simulink model "EvitarObstaculo_traj"  (R2023b)
settings: Solver=FixedStepAuto  StartTime=0.0  StopTime=100.0  FixedStep=Ts  RelTol=1e-3
values from neighbouring files (symbols this model uses):
  obsx = 2    [EjecutarEsquivarObs.m]    (also in EjecutarEsquivarObs_traj.m = 1.75)
  obsy = 0    [EjecutarEsquivarObs.m]    (also in EjecutarEsquivarObs_traj.m = 0.7)
  th_0 = 0    [EjecutarBorroso_traj.m]    (also in EjecutarEsquivarObs_traj.m)
  Ts = 100e-3    (= 0.1)    [EjecutarBorroso.m]    (also in EjecutarBorroso_traj.m; EjecutarEsquivarObs.m; EjecutarEsquivarObs_traj.m)
  x_0 = 0.1    [EjecutarBorroso_traj.m]    (also in EjecutarEsquivarObs_traj.m)
  y_0 = 0    [EjecutarBorroso_traj.m]    (also in EjecutarEsquivarObs_traj.m)
undefined symbols (not defined in the file or in its folder): DiscIntNeverNeededParam, sigbuilder_block
libraries: fuzblock x1
settings Model: Creator=perez  LastModifiedBy=perez
settings DataIOCC: ReturnWorkspaceOutputs=off

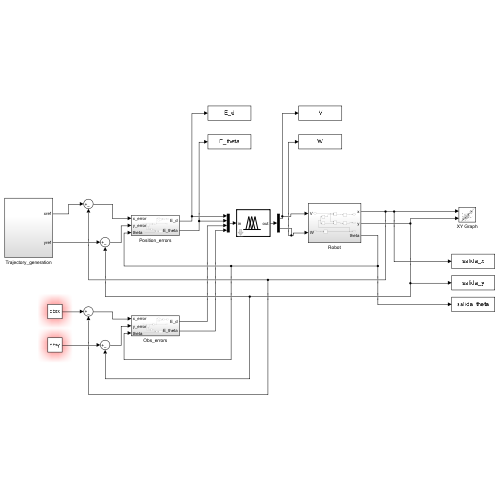
[thumbnail: Simulink's stored preview of the top-level diagram]
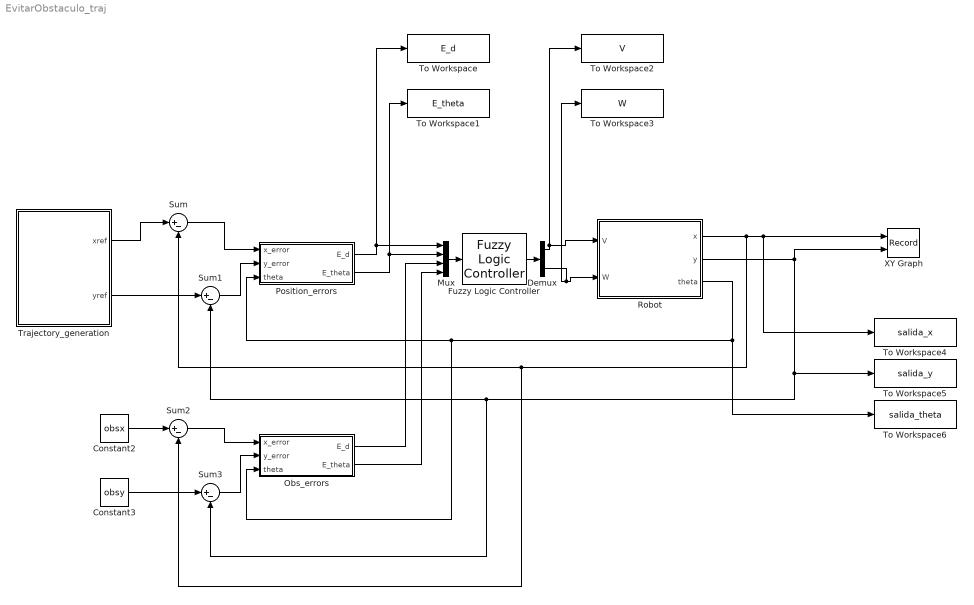
== system EvitarObstaculo_traj ==
  Constant2 : Constant  Value=obsx
  Constant3 : Constant  Value=obsy
  Demux : Demux  Outputs=2
  Fuzzy Logic Controller : fuzblock/Fuzzy Logic  Controller  FIS='ControlBorrosoObs.fis'  OutputSampleNumber=101  DataType=double  FuzzifiedInputs=off  RuleFiringStrengths=off  RuleOutputs=off  AggregatedOutputs=off  SimulateUsing=Interpreted execution  OutOfRangeInputValueMessage=warning  NoRuleFiredMessage=warning  EmptyOutputFuzzySetMessage=warning
  Mux : Mux
  Obs_errors : Subsystem
  Position_errors : Subsystem
  Robot : Subsystem
  Sum{,1..3} (4 alike) : Sum  Inputs=|+-
  To Workspace : ToWorkspace  VariableName=E_d  SaveFormat=Structure With Time  SampleTime=-1
  To Workspace1 : ToWorkspace  VariableName=E_theta  SaveFormat=Structure With Time  SampleTime=-1
  To Workspace2 : ToWorkspace  VariableName=V  SaveFormat=Structure With Time  SampleTime=-1
  To Workspace3 : ToWorkspace  VariableName=W  SaveFormat=Structure With Time  SampleTime=-1
  To Workspace4 : ToWorkspace  VariableName=salida_x  SaveFormat=Structure With Time  SampleTime=-1
  To Workspace5 : ToWorkspace  VariableName=salida_y  SaveFormat=Structure With Time  SampleTime=-1
  To Workspace6 : ToWorkspace  VariableName=salida_theta  SaveFormat=Structure With Time  SampleTime=-1
  Trajectory_generation : Subsystem
  XY Graph : Record  FileSettingsInternal="{\"entries\":[{\"content\":{\"excelSettings\":{\"content\":{},\"type\":\"Streamout.ExcelSettings\"}},\"type\":\"Streamout.FileSettingStorage\",\"uuid\":\"\"}],\"packageUris\":[\"http:\\/\\/schema.mathworks.com\\/mf0\\/streamout_blocks\\/R2020a\"],\"version\":\"1.0\"}"  Layout=[1 1]  SignalsInternal="{\"entries\":[{\"content\":{\"signals\":[{\"content\":{\"blockPath\":[],\"dimensions\":[1],\"domain\":\"\",\"lineColor\":\"#a2142f\",\"plots\":[ 1 ],\"port\":1,\"signalID\":1,\"signalName\":\"Robot:1\"},\"type\":\"RecordBlkView.Signal\",\"uuid\":\"\"},{\"content\":{\"blockPath\":[],\"dimensions\":[1],\"domain\":\"\",\"lineColor\":\"#139fff\",\"plots\":[ 1 ],\"port\":2,\"signalID\":2,\"signalName\":\"Robot:2\"},\"type\":\"RecordBlkView.Signal\",\"uuid\":\"\"}]},\"type\":\"RecordBlkView.InputSignals\",\"uuid\":\"\"}],\"packageUris\":[\"http:\\/\\/schema.mathworks.com\\/mf0\\/streamout_blocks\\/R2020a\"],\"version\":\"1.0\"}"  VisualizationBindings="{\"xyplotplugin\":{\"info\":[{\"series\":[{\"bindingParametersList\":[{\"parameter\":\"X-Axis\",\"signalID\":1,\"signalName\":\"Robot:1\"},{\"parameter\":\"Y-Axis\",\"signalID\":2,\"signalName\":\"Robot:2\"}],\"seriesID\":0}],\"subplotID\":1}]}}"  CompatibilityTag=XY
  wires:
  Trajectory_generation/1(xref) -> Sum/1
  Sum/1 -> Position_errors/1(x_error)
  Sum1/1 -> Position_errors/2(y_error)
  Position_errors/1(E_d) -> Mux/1, To Workspace/1
  Position_errors/2(E_theta) -> Mux/2, To Workspace1/1
  Demux/1 -> To Workspace2/1, Robot/1(V)
  Demux/2 -> To Workspace3/1, Robot/2(W)
  Robot/1(x) -> Sum2/2, Sum/2, To Workspace4/1, XY Graph/1
  Robot/2(y) -> To Workspace5/1, Sum3/2, Sum1/2, XY Graph/2
  Robot/3(theta) -> To Workspace6/1, Obs_errors/3(theta), Position_errors/3(theta)
  Trajectory_generation/2(yref) -> Sum1/1
  Mux/1 -> Fuzzy Logic Controller/1
  Fuzzy Logic Controller/1 -> Demux/1
  Constant2/1 -> Sum2/1
  Constant3/1 -> Sum3/1
  Sum2/1 -> Obs_errors/1(x_error)
  Sum3/1 -> Obs_errors/2(y_error)
  Obs_errors/1(E_d) -> Mux/3
  Obs_errors/2(E_theta) -> Mux/4

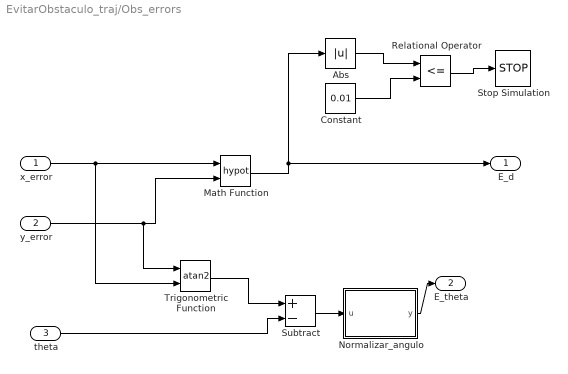
== system EvitarObstaculo_traj/Obs_errors ==
  x_error : Inport
  y_error : Inport  Port=2
  theta : Inport  Port=3
  Abs : Abs  SaturateOnIntegerOverflow=off
  Constant : Constant  Value=0.01
  Math Function : Math  Operator=hypot
  Normalizar_angulo : MATLAB Function  TreatAsAtomicUnit=on
  Relational Operator : RelationalOperator  Operator=<=  OutDataTypeStr=boolean  RndMeth=Simplest  InputSameDT=off
  Stop Simulation : Stop
  Subtract : Sum  Inputs=+-
  Trigonometric Function : Trigonometry  Operator=atan2
  E_d : Outport
  E_theta : Outport  Port=2
  wires:
  x_error/1 -> Trigonometric Function/2, Math Function/1
  y_error/1 -> Trigonometric Function/1, Math Function/2
  Trigonometric Function/1 -> Subtract/1
  theta/1 -> Subtract/2
  Subtract/1 -> Normalizar_angulo/1(u)
  Normalizar_angulo/1(y) -> E_theta/1
  Abs/1 -> Relational Operator/1
  Constant/1 -> Relational Operator/2
  Math Function/1 -> E_d/1, Abs/1
  Relational Operator/1 -> Stop Simulation/1

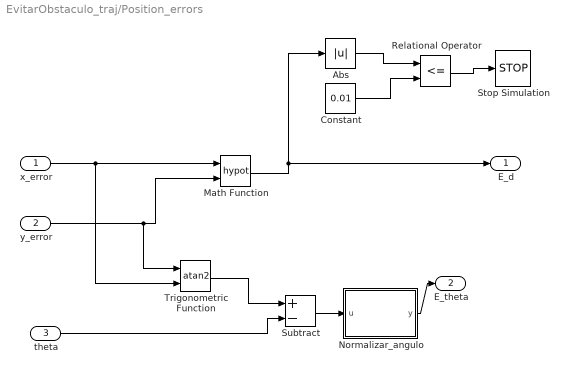
== system EvitarObstaculo_traj/Position_errors ==
  x_error : Inport
  y_error : Inport  Port=2
  theta : Inport  Port=3
  Abs : Abs  SaturateOnIntegerOverflow=off
  Constant : Constant  Value=0.01
  Math Function : Math  Operator=hypot
  Normalizar_angulo : MATLAB Function  TreatAsAtomicUnit=on
  Relational Operator : RelationalOperator  Operator=<=  OutDataTypeStr=boolean  RndMeth=Simplest  InputSameDT=off
  Stop Simulation : Stop
  Subtract : Sum  Inputs=+-
  Trigonometric Function : Trigonometry  Operator=atan2
  E_d : Outport
  E_theta : Outport  Port=2
  wires:
  x_error/1 -> Trigonometric Function/2, Math Function/1
  y_error/1 -> Trigonometric Function/1, Math Function/2
  Trigonometric Function/1 -> Subtract/1
  theta/1 -> Subtract/2
  Subtract/1 -> Normalizar_angulo/1(u)
  Normalizar_angulo/1(y) -> E_theta/1
  Abs/1 -> Relational Operator/1
  Constant/1 -> Relational Operator/2
  Math Function/1 -> E_d/1, Abs/1
  Relational Operator/1 -> Stop Simulation/1

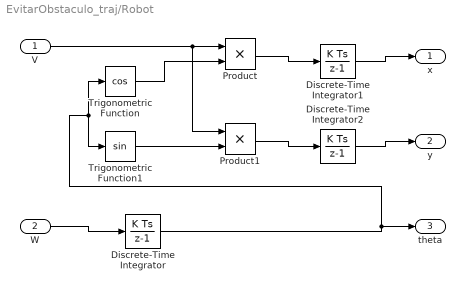
== system EvitarObstaculo_traj/Robot ==
  V : Inport
  W : Inport  Port=2
  Discrete-Time Integrator : DiscreteIntegrator  SampleTime=-1  ICPrevOutput=DiscIntNeverNeededParam  ICPrevScaledInput=DiscIntNeverNeededParam
  Discrete-Time Integrator1 : DiscreteIntegrator  SampleTime=-1  ICPrevOutput=DiscIntNeverNeededParam  ICPrevScaledInput=DiscIntNeverNeededParam
  Discrete-Time Integrator2 : DiscreteIntegrator  SampleTime=-1  ICPrevOutput=DiscIntNeverNeededParam  ICPrevScaledInput=DiscIntNeverNeededParam
  Product : Product
  Product1 : Product
  Trigonometric Function : Trigonometry  Operator=cos
  Trigonometric Function1 : Trigonometry
  x : Outport
  y : Outport  Port=2
  theta : Outport  Port=3
  wires:
  Trigonometric Function1/1 -> Product1/2
  Discrete-Time Integrator2/1 -> y/1
  Discrete-Time Integrator1/1 -> x/1
  Product/1 -> Discrete-Time Integrator1/1
  Product1/1 -> Discrete-Time Integrator2/1
  V/1 -> Product1/1, Product/1
  Discrete-Time Integrator/1 -> Trigonometric Function1/1, Trigonometric Function/1, theta/1
  Trigonometric Function/1 -> Product/2
  W/1 -> Discrete-Time Integrator/1

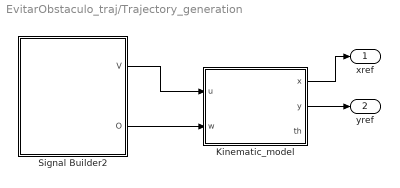
== system EvitarObstaculo_traj/Trajectory_generation ==
  Kinematic_model : Subsystem
  Signal Builder2 : Subsystem  Tag=STV Subsys  LoadFcn=sigbuilder_block('load');  StartFcn=sigbuilder_block('start');  StopFcn=sigbuilder_block('stop');  ClipboardFcn=sigbuilder_block('clipboard');  mask(Sigbuilder block){tuvar=[0:10]}
      mask help: Sigbuilder GUI
      mask init:
      | if ~strcmp(get_param(bdroot(gcbh),'SimulationStatus'),'stopped') tuvar = sigbuilder_block('maskInit'); end
      settings: CopyFcn=sigbuilder_block('copy');  DeleteFcn=sigbuilder_block('delete');  ModelCloseFcn=sigbuilder_block('modelClose');  PreSaveFcn=sigbuilder_block('preSave');  PauseFcn=sigbuilder_block('pause')  ContinueFcn=sigbuilder_block('continue')  NameChangeFcn=sigbuilder_block('namechange');  OpenFcn=sigbuilder_block('open',[60 82.4 534.4 508 ]);  CloseFcn=sigbuilder_block('close');
      mask Display: plot(0, 0, 100, 100,[2, 2, 32, 32, 2], [68, 8, 8, 68, 68],[32, 2], [38, 38], [32, 19, 2],[53, 60, 44], [32, 17, 17, 2],[16, 16, 31, 31]);txt = getActiveGroup(gcbh);text(2, 100, txt,'verticalAlignment', 'top');
  xref : Outport  VectorParamsAs1DForOutWhenUnconnected=off
  yref : Outport  Port=2  VectorParamsAs1DForOutWhenUnconnected=off
  wires:
  Signal Builder2/1(V) -> Kinematic_model/1(u)
  Signal Builder2/2(O) -> Kinematic_model/2(w)
  Kinematic_model/1(x) -> xref/1
  Kinematic_model/2(y) -> yref/1

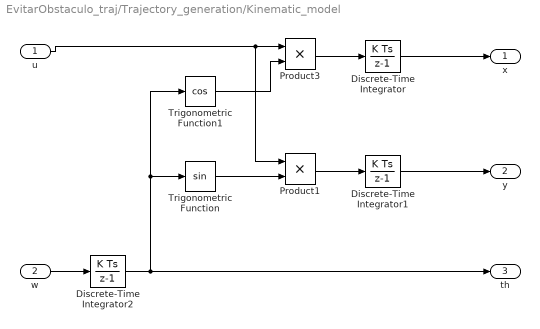
== system EvitarObstaculo_traj/Trajectory_generation/Kinematic_model ==
  u : Inport
  w : Inport  Port=2
  Discrete-Time Integrator : DiscreteIntegrator  InitialCondition=x_0  SampleTime=Ts  ICPrevOutput=DiscIntNeverNeededParam  ICPrevScaledInput=DiscIntNeverNeededParam
  Discrete-Time Integrator1 : DiscreteIntegrator  InitialCondition=y_0  SampleTime=Ts  ICPrevOutput=DiscIntNeverNeededParam  ICPrevScaledInput=DiscIntNeverNeededParam
  Discrete-Time Integrator2 : DiscreteIntegrator  InitialCondition=th_0  SampleTime=Ts  ICPrevOutput=DiscIntNeverNeededParam  ICPrevScaledInput=DiscIntNeverNeededParam
  Product1 : Product
  Product3 : Product
  Trigonometric Function : Trigonometry
  Trigonometric Function1 : Trigonometry  Operator=cos
  x : Outport  VectorParamsAs1DForOutWhenUnconnected=off
  y : Outport  Port=2  VectorParamsAs1DForOutWhenUnconnected=off
  th : Outport  Port=3  VectorParamsAs1DForOutWhenUnconnected=off
  wires:
  Discrete-Time Integrator2/1 -> Trigonometric Function1/1, Trigonometric Function/1, th/1
  Product1/1 -> Discrete-Time Integrator1/1
  Product3/1 -> Discrete-Time Integrator/1
  w/1 -> Discrete-Time Integrator2/1
  Trigonometric Function/1 -> Product1/2
  u/1 -> Product1/1, Product3/1
  Trigonometric Function1/1 -> Product3/2
  Discrete-Time Integrator1/1 -> y/1
  Discrete-Time Integrator/1 -> x/1

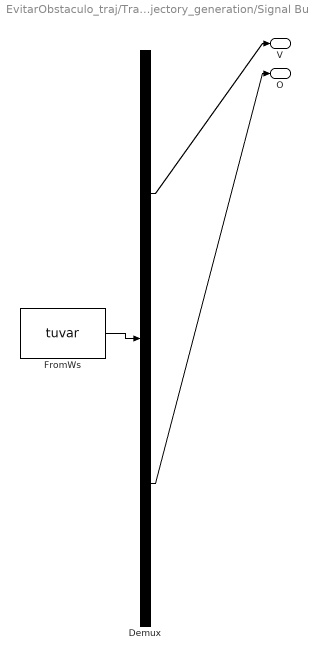
== system EvitarObstaculo_traj/Trajectory_generation/Signal Builder2 ==
  Demux : Demux  Tag=STV Demux  Outputs=2
      settings: DisplayOption=none
  FromWs : FromWorkspace  Tag=STV FromWs  VariableName=tuvar
      SigBuilderData=|
      | common.afterFinalStr = 'Extrapolate'
      | common.sampleTime = '0'
      | dataSet.timeRange = [0 115]
      | dataSet.name = 'Group 1'
      | sbobj.Groups.Name = 'Group 1'
      | sbobj.Groups.Signals(1).Name = 'V'
      | sbobj.Groups.Signals(1).XData = [0 87 87 115]
      | sbobj.Groups.Signals(1).YData = [0.25 0.25 0 0]
      | sbobj.Groups.Signals(2).Name = 'O'
      | sbobj.Groups.Signals(2).XData = [0 12 12 30.849 30.849 55.981 55.981 74.83 74.83 99.962 115]
      | sbobj.Groups.Signals(2).YData = [0 0 0.25 0.25 -0.25 -0.25 0.25 0.25 0 0 0]
      | sbobj.Groups.TimeRange = [0 115]
  V : Outport  Tag=STV Outport  VectorParamsAs1DForOutWhenUnconnected=off
  O : Outport  Tag=STV Outport  Port=2  VectorParamsAs1DForOutWhenUnconnected=off
  wires:
  FromWs/1 -> Demux/1
  Demux/1 -> V/1
  Demux/2 -> O/1

== matlab function EvitarObstaculo_traj/Position_errors/Normalizar_angulo ==
  data: u input; y output
function y = fcn(u)
% Lleva el ángulo u (rad) a su equivalente en [-pi, pi):
% +pi pasa el intervalo a [0, 2pi), mod quita las vueltas completas
% (también con u negativo) y -pi lo devuelve al intervalo original
y = mod(u + pi, 2*pi) - pi;

== matlab function EvitarObstaculo_traj/Obs_errors/Normalizar_angulo ==
  data: u input; y output
function y = fcn(u)
% Lleva el ángulo u (rad) a su equivalente en [-pi, pi):
% +pi pasa el intervalo a [0, 2pi), mod quita las vueltas completas
% (también con u negativo) y -pi lo devuelve al intervalo original
y = mod(u + pi, 2*pi) - pi;
